simulink model "macroRobot_simulator"  (R2025a)
settings: Solver=FixedStepAuto  StartTime=0.0  StopTime=120  FixedStep=TsControl  MaxStep=0.00025  RelTol=1e-3
PreLoadFcn:
  | initMacroRobotSimulator;
InitFcn:
  | initMacroRobotSimulator;
values from neighbouring files (symbols this model uses):
  initState = deg2rad([-109; +67; +71; -111; -59; +20; -18])    [initMacroRobotSimulator.m]
undefined symbols (not defined in the file or in its folder): smiData, T_b_LaserGate, T_F1_Center, T_F1_Square1, T_F1_Square2, T_F1_Z1, T_F1_Z2, TsControl, X, Y, Z
libraries: sm_lib x50, nesl_utility x13, simulink x1, matrix_library x1, lib_lowLevelController x1, lib_ForwardKinematicsMacroRobot x1, lib_highLevelController x1, lib_InverseKinematicsMacroRobotVelocity x1, lib_saturateMacroRobotPosition x1
(part 2 of 2)

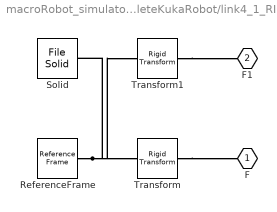
== system macroRobot_simulator/Simulation/completeKukaRobot/link4_1_RIGID ==
  ReferenceFrame : sm_lib/Frames and Transforms/Reference Frame
  Solid : sm_lib/Body Elements/File Solid  ExtGeomFileName=link4_Default_sldprt.STEP  UnitType=FromFile  ExtGeomFileUnits=m  StepReaderType=HEX  ExportConvexHullGeometry=off  InertiaType=Custom  BasedOnType=DensityFromFile  Density=1000  DensityUnits=kg/m^3  Mass=smiData.Solid(4).mass  MassUnits=kg  CenterOfMass=smiData.Solid(4).CoM  CenterOfMassUnits=mm  MomentsOfInertia=smiData.Solid(4).MoI  MomentsOfInertiaUnits=kg*mm^2  ProductsOfInertia=smiData.Solid(4).PoI  ProductsOfInertiaUnits=kg*mm^2  GraphicType=FromGeometry  MarkerShape=Sphere  MarkerSize=10  GraphicVisPropType=SimpleVisualProperties  GraphicDiffuseColor=smiData.Solid(4).color  GraphicOpacity=smiData.Solid(4).opacity  GraphicSpecularColor=[0.5 0.5 0.5 1.0]  GraphicAmbientColor=[0.15 0.15 0.15 1.0]  GraphicEmissiveColor=[0.0 0.0 0.0 1.0]  GraphicShininess=75  DoExposeReferenceFrame=on  SerializedFrames=<Frames/>
  Transform : sm_lib/Frames and Transforms/Rigid Transform  RotationMethod=ArbitraryAxis  FollAlignAxisA=+X  BaseAlignAxisA=+Y  FollAlignAxisB=+Y  BaseAlignAxisB=+Z  RotationStandardAxis=+Z  RotationAngle=smiData.RigidTransform(8).angle  RotationAngleUnits=rad  RotationArbitraryAxis=smiData.RigidTransform(8).axis  RotationSequenceAxes=FollowerAxes  RotationSequence=XYX  RotationSequenceAngles=[0 0 0]  RotationSequenceAnglesUnits=deg  RotationMatrix=[1 0 0; 0 1 0; 0 0 1]  Quaternion=[1 0 0 0]  TranslationMethod=Cartesian  TranslationCartesianOffset=smiData.RigidTransform(8).translation  TranslationCartesianOffsetUnits=mm  TranslationStandardAxis=+Z  TranslationStandardOffset=0  TranslationStandardOffsetUnits=m  TranslationROffset=0  TranslationROffsetUnits=m  TranslationThetaOffset=0  TranslationThetaOffsetUnits=deg  TranslationZOffset=0  TranslationZOffsetUnits=m
  Transform1 : sm_lib/Frames and Transforms/Rigid Transform  RotationMethod=ArbitraryAxis  FollAlignAxisA=+X  BaseAlignAxisA=+Y  FollAlignAxisB=+Y  BaseAlignAxisB=+Z  RotationStandardAxis=+Z  RotationAngle=smiData.RigidTransform(9).angle  RotationAngleUnits=rad  RotationArbitraryAxis=smiData.RigidTransform(9).axis  RotationSequenceAxes=FollowerAxes  RotationSequence=XYX  RotationSequenceAngles=[0 0 0]  RotationSequenceAnglesUnits=deg  RotationMatrix=[1 0 0; 0 1 0; 0 0 1]  Quaternion=[1 0 0 0]  TranslationMethod=Cartesian  TranslationCartesianOffset=smiData.RigidTransform(9).translation  TranslationCartesianOffsetUnits=mm  TranslationStandardAxis=+Z  TranslationStandardOffset=0  TranslationStandardOffsetUnits=m  TranslationROffset=0  TranslationROffsetUnits=m  TranslationThetaOffset=0  TranslationThetaOffsetUnits=deg  TranslationZOffset=0  TranslationZOffsetUnits=m
  F : PMIOPort  Side=Left
  F1 : PMIOPort  Port=2  Side=Right
  connections:
  ReferenceFrame/RConn1 -- Solid/RConn1 -- Transform/LConn1 -- Transform1/LConn1
  Transform/RConn1 -- F/RConn1
  Transform1/RConn1 -- F1/RConn1

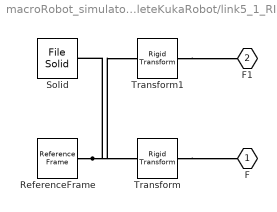
== system macroRobot_simulator/Simulation/completeKukaRobot/link5_1_RIGID ==
  ReferenceFrame : sm_lib/Frames and Transforms/Reference Frame
  Solid : sm_lib/Body Elements/File Solid  ExtGeomFileName=link5_Default_sldprt.STEP  UnitType=FromFile  ExtGeomFileUnits=m  StepReaderType=HEX  ExportConvexHullGeometry=off  InertiaType=Custom  BasedOnType=DensityFromFile  Density=1000  DensityUnits=kg/m^3  Mass=smiData.Solid(5).mass  MassUnits=kg  CenterOfMass=smiData.Solid(5).CoM  CenterOfMassUnits=mm  MomentsOfInertia=smiData.Solid(5).MoI  MomentsOfInertiaUnits=kg*mm^2  ProductsOfInertia=smiData.Solid(5).PoI  ProductsOfInertiaUnits=kg*mm^2  GraphicType=FromGeometry  MarkerShape=Sphere  MarkerSize=10  GraphicVisPropType=SimpleVisualProperties  GraphicDiffuseColor=smiData.Solid(5).color  GraphicOpacity=smiData.Solid(5).opacity  GraphicSpecularColor=[0.5 0.5 0.5 1.0]  GraphicAmbientColor=[0.15 0.15 0.15 1.0]  GraphicEmissiveColor=[0.0 0.0 0.0 1.0]  GraphicShininess=75  DoExposeReferenceFrame=on  SerializedFrames=<Frames/>
  Transform : sm_lib/Frames and Transforms/Rigid Transform  RotationMethod=ArbitraryAxis  FollAlignAxisA=+X  BaseAlignAxisA=+Y  FollAlignAxisB=+Y  BaseAlignAxisB=+Z  RotationStandardAxis=+Z  RotationAngle=smiData.RigidTransform(10).angle  RotationAngleUnits=rad  RotationArbitraryAxis=smiData.RigidTransform(10).axis  RotationSequenceAxes=FollowerAxes  RotationSequence=XYX  RotationSequenceAngles=[0 0 0]  RotationSequenceAnglesUnits=deg  RotationMatrix=[1 0 0; 0 1 0; 0 0 1]  Quaternion=[1 0 0 0]  TranslationMethod=Cartesian  TranslationCartesianOffset=smiData.RigidTransform(10).translation  TranslationCartesianOffsetUnits=mm  TranslationStandardAxis=+Z  TranslationStandardOffset=0  TranslationStandardOffsetUnits=m  TranslationROffset=0  TranslationROffsetUnits=m  TranslationThetaOffset=0  TranslationThetaOffsetUnits=deg  TranslationZOffset=0  TranslationZOffsetUnits=m
  Transform1 : sm_lib/Frames and Transforms/Rigid Transform  RotationMethod=ArbitraryAxis  FollAlignAxisA=+X  BaseAlignAxisA=+Y  FollAlignAxisB=+Y  BaseAlignAxisB=+Z  RotationStandardAxis=+Z  RotationAngle=smiData.RigidTransform(11).angle  RotationAngleUnits=rad  RotationArbitraryAxis=smiData.RigidTransform(11).axis  RotationSequenceAxes=FollowerAxes  RotationSequence=XYX  RotationSequenceAngles=[0 0 0]  RotationSequenceAnglesUnits=deg  RotationMatrix=[1 0 0; 0 1 0; 0 0 1]  Quaternion=[1 0 0 0]  TranslationMethod=Cartesian  TranslationCartesianOffset=smiData.RigidTransform(11).translation  TranslationCartesianOffsetUnits=mm  TranslationStandardAxis=+Z  TranslationStandardOffset=0  TranslationStandardOffsetUnits=m  TranslationROffset=0  TranslationROffsetUnits=m  TranslationThetaOffset=0  TranslationThetaOffsetUnits=deg  TranslationZOffset=0  TranslationZOffsetUnits=m
  F : PMIOPort  Side=Left
  F1 : PMIOPort  Port=2  Side=Right
  connections:
  ReferenceFrame/RConn1 -- Solid/RConn1 -- Transform/LConn1 -- Transform1/LConn1
  Transform/RConn1 -- F/RConn1
  Transform1/RConn1 -- F1/RConn1

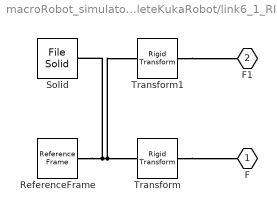
== system macroRobot_simulator/Simulation/completeKukaRobot/link6_1_RIGID ==
  ReferenceFrame : sm_lib/Frames and Transforms/Reference Frame
  Solid : sm_lib/Body Elements/File Solid  ExtGeomFileName=link6_Default_sldprt.STEP  UnitType=FromFile  ExtGeomFileUnits=m  StepReaderType=HEX  ExportConvexHullGeometry=off  InertiaType=Custom  BasedOnType=DensityFromFile  Density=1000  DensityUnits=kg/m^3  Mass=smiData.Solid(8).mass  MassUnits=kg  CenterOfMass=smiData.Solid(8).CoM  CenterOfMassUnits=mm  MomentsOfInertia=smiData.Solid(8).MoI  MomentsOfInertiaUnits=kg*mm^2  ProductsOfInertia=smiData.Solid(8).PoI  ProductsOfInertiaUnits=kg*mm^2  GraphicType=FromGeometry  MarkerShape=Sphere  MarkerSize=10  GraphicVisPropType=SimpleVisualProperties  GraphicDiffuseColor=smiData.Solid(8).color  GraphicOpacity=smiData.Solid(8).opacity  GraphicSpecularColor=[0.5 0.5 0.5 1.0]  GraphicAmbientColor=[0.15 0.15 0.15 1.0]  GraphicEmissiveColor=[0.0 0.0 0.0 1.0]  GraphicShininess=75  DoExposeReferenceFrame=on  SerializedFrames=<Frames/>
  Transform : sm_lib/Frames and Transforms/Rigid Transform  RotationMethod=ArbitraryAxis  FollAlignAxisA=+X  BaseAlignAxisA=+Y  FollAlignAxisB=+Y  BaseAlignAxisB=+Z  RotationStandardAxis=+Z  RotationAngle=smiData.RigidTransform(12).angle  RotationAngleUnits=rad  RotationArbitraryAxis=smiData.RigidTransform(12).axis  RotationSequenceAxes=FollowerAxes  RotationSequence=XYX  RotationSequenceAngles=[0 0 0]  RotationSequenceAnglesUnits=deg  RotationMatrix=[1 0 0; 0 1 0; 0 0 1]  Quaternion=[1 0 0 0]  TranslationMethod=Cartesian  TranslationCartesianOffset=smiData.RigidTransform(12).translation  TranslationCartesianOffsetUnits=mm  TranslationStandardAxis=+Z  TranslationStandardOffset=0  TranslationStandardOffsetUnits=m  TranslationROffset=0  TranslationROffsetUnits=m  TranslationThetaOffset=0  TranslationThetaOffsetUnits=deg  TranslationZOffset=0  TranslationZOffsetUnits=m
  Transform1 : sm_lib/Frames and Transforms/Rigid Transform  RotationMethod=ArbitraryAxis  FollAlignAxisA=+X  BaseAlignAxisA=+Y  FollAlignAxisB=+Y  BaseAlignAxisB=+Z  RotationStandardAxis=+Z  RotationAngle=smiData.RigidTransform(13).angle  RotationAngleUnits=rad  RotationArbitraryAxis=smiData.RigidTransform(13).axis  RotationSequenceAxes=FollowerAxes  RotationSequence=XYX  RotationSequenceAngles=[0 0 0]  RotationSequenceAnglesUnits=deg  RotationMatrix=[1 0 0; 0 1 0; 0 0 1]  Quaternion=[1 0 0 0]  TranslationMethod=Cartesian  TranslationCartesianOffset=smiData.RigidTransform(13).translation  TranslationCartesianOffsetUnits=mm  TranslationStandardAxis=+Z  TranslationStandardOffset=0  TranslationStandardOffsetUnits=m  TranslationROffset=0  TranslationROffsetUnits=m  TranslationThetaOffset=0  TranslationThetaOffsetUnits=deg  TranslationZOffset=0  TranslationZOffsetUnits=m
  F : PMIOPort  Side=Left
  F1 : PMIOPort  Port=2  Side=Right
  connections:
  ReferenceFrame/RConn1 -- Transform/LConn1 -- Transform1/LConn1 -- Solid/RConn1
  Transform/RConn1 -- F/RConn1
  Transform1/RConn1 -- F1/RConn1

== system macroRobot_simulator/Simulation/completeKukaRobot/link7_1_RIGID ==
  ReferenceFrame : sm_lib/Frames and Transforms/Reference Frame
  Solid : sm_lib/Body Elements/File Solid  ExtGeomFileName=link7_Default_sldprt.STEP  UnitType=FromFile  ExtGeomFileUnits=m  StepReaderType=HEX  ExportConvexHullGeometry=off  InertiaType=Custom  BasedOnType=DensityFromFile  Density=1000  DensityUnits=kg/m^3  Mass=smiData.Solid(1).mass  MassUnits=kg  CenterOfMass=smiData.Solid(1).CoM  CenterOfMassUnits=mm  MomentsOfInertia=smiData.Solid(1).MoI  MomentsOfInertiaUnits=kg*mm^2  ProductsOfInertia=smiData.Solid(1).PoI  ProductsOfInertiaUnits=kg*mm^2  GraphicType=FromGeometry  MarkerShape=Sphere  MarkerSize=10  GraphicVisPropType=SimpleVisualProperties  GraphicDiffuseColor=smiData.Solid(1).color  GraphicOpacity=smiData.Solid(1).opacity  GraphicSpecularColor=[0.5 0.5 0.5 1.0]  GraphicAmbientColor=[0.15 0.15 0.15 1.0]  GraphicEmissiveColor=[0.0 0.0 0.0 1.0]  GraphicShininess=75  DoExposeReferenceFrame=on  SerializedFrames=<Frames><Frame><Id>Frame1</Id><Value><Name>F1</Name><Origin><Source>GeometricFeature</Source><FeatureName>planar surface 30</FeatureName></Origin><PrimaryAxis><DefinedDirection>+Z</DefinedDirection><Source>ReferenceFrame</Source><SourceDirection>+Z</SourceDirection><FeatureName></FeatureName></PrimaryAxis><SecondaryAxis><DefinedDirection>+X</DefinedDirection><Source>ReferenceFrame</Source><SourceDirection>+X</SourceDirection><FeatureName></FeatureName></SecondaryAxis></Value></Frame></Frames>
  Transform : sm_lib/Frames and Transforms/Rigid Transform  RotationMethod=ArbitraryAxis  FollAlignAxisA=+X  BaseAlignAxisA=+Y  FollAlignAxisB=+Y  BaseAlignAxisB=+Z  RotationStandardAxis=+Z  RotationAngle=smiData.RigidTransform(14).angle  RotationAngleUnits=rad  RotationArbitraryAxis=smiData.RigidTransform(14).axis  RotationSequenceAxes=FollowerAxes  RotationSequence=XYX  RotationSequenceAngles=[0 0 0]  RotationSequenceAnglesUnits=deg  RotationMatrix=[1 0 0; 0 1 0; 0 0 1]  Quaternion=[1 0 0 0]  TranslationMethod=Cartesian  TranslationCartesianOffset=smiData.RigidTransform(14).translation  TranslationCartesianOffsetUnits=mm  TranslationStandardAxis=+Z  TranslationStandardOffset=0  TranslationStandardOffsetUnits=m  TranslationROffset=0  TranslationROffsetUnits=m  TranslationThetaOffset=0  TranslationThetaOffsetUnits=deg  TranslationZOffset=0  TranslationZOffsetUnits=m
  F : PMIOPort  Side=Left
  F1 : PMIOPort  Port=2  Side=Right
  connections:
  ReferenceFrame/RConn1 -- Solid/RConn1 -- Transform/LConn1
  Transform/RConn1 -- F/RConn1
  F1/RConn1 -- Solid/LConn1

== system macroRobot_simulator/Simulation/completeKukaRobot/tool ==
  File Solid : sm_lib/Body Elements/File Solid  ExtGeomFileName=/home/gordi/Documentos/Máster/BASILEA/3rd Semester/A. Medical Robotics/Project/codeBaseSimulator/Library/Visualizer/20261016_extruder_mockup.STEP  UnitType=FromFile  ExtGeomFileUnits=m  StepReaderType=HEX  ExportConvexHullGeometry=off  InertiaType=PointMass  BasedOnType=DensityFromFile  Density=1000  DensityUnits=kg/m^3  Mass=1  MassUnits=kg  CenterOfMass=[0 0 0]  CenterOfMassUnits=m  MomentsOfInertia=[1 1 1]  MomentsOfInertiaUnits=kg*m^2  ProductsOfInertia=[0 0 0]  ProductsOfInertiaUnits=kg*m^2  GraphicType=FromGeometry  MarkerShape=Sphere  MarkerSize=10  GraphicVisPropType=SimpleVisualProperties  GraphicDiffuseColor=[0.5 0.5 0.5]  GraphicOpacity=1  GraphicSpecularColor=[0.5 0.5 0.5 1.0]  GraphicAmbientColor=[0.15 0.15 0.15 1.0]  GraphicEmissiveColor=[0.0 0.0 0.0 1.0]  GraphicShininess=75  DoExposeReferenceFrame=off  SerializedFrames=<Frames><Frame><Id>Frame1</Id><Value><Name>F1</Name><Origin><Source>GeometricFeature</Source><FeatureName>planar surface 33</FeatureName></Origin><PrimaryAxis><DefinedDirection>-Z</DefinedDirection><Source>GeometricFeature</Source><SourceDirection>+Y</SourceDirection><FeatureName>segment 40</FeatureName></PrimaryAxis><SecondaryAxis><DefinedDirection>+X</DefinedDirection><Source>GeometricFeature</Source><SourceDirection>+Z</SourceDirection><FeatureName>segment 53</FeatureName></SecondaryAxis></Value></Frame><Frame><Id>Frame2</Id><Value><Name>F2</Name><Origin><Source>GeometricFeature</Source><FeatureName>planar surface 266</FeatureName></Origin><PrimaryAxis><DefinedDirection>+Z</DefinedDirection><Source>ReferenceFrame</Source><SourceDirection>-Y</SourceDirection><FeatureName></FeatureName></PrimaryAxis><SecondaryAxis><DefinedDirection>+X</DefinedDirection><Source>ReferenceFrame</Source><SourceDirection>-Z</SourceDirection><FeatureName></FeatureName></SecondaryAxis></Value></Frame></Frames>
  ReferenceFrame : sm_lib/Frames and Transforms/Reference Frame
  Transform1 : sm_lib/Frames and Transforms/Rigid Transform  Commented=on  RotationMethod=RotationMatrix  FollAlignAxisA=+X  BaseAlignAxisA=+Y  FollAlignAxisB=+Y  BaseAlignAxisB=+Z  RotationStandardAxis=+Z  RotationAngle=smiData.RigidTransform(14).angle  RotationAngleUnits=rad  RotationArbitraryAxis=smiData.RigidTransform(14).axis  RotationSequenceAxes=FollowerAxes  RotationSequence=XYX  RotationSequenceAngles=[0 0 0]  RotationSequenceAnglesUnits=deg  RotationMatrix=[cos(pi/4) 0 -sin(pi/4); 0 1 0; sin(pi/4) 0 cos(pi/4)]  Quaternion=[1 0 0 0]  TranslationMethod=Cartesian  TranslationCartesianOffset=[0.0462 0 0.1452]  TranslationCartesianOffsetUnits=mm  TranslationStandardAxis=+Z  TranslationStandardOffset=0  TranslationStandardOffsetUnits=m  TranslationROffset=0  TranslationROffsetUnits=m  TranslationThetaOffset=0  TranslationThetaOffsetUnits=deg  TranslationZOffset=0  TranslationZOffsetUnits=m
  F1 : PMIOPort  Side=Left
  F2 : PMIOPort  Port=2  Side=Right
  connections:
  ReferenceFrame/RConn1 -- F1/RConn1 -- File Solid/LConn1
  File Solid/RConn1 -- F2/RConn1

== matlab function macroRobot_simulator/Simulation/completeKukaRobot/MATLAB Function ==
  data: commandedJoints input; jointsForModel output
function jointsForModel  = jointOrientationToModel(commandedJoints)


jointsForModel = commandedJoints(1:7);
jointsForModel([3,4,5,6,7]) = -commandedJoints([3,4,5,6,7]);
%joints(5) = -u(5);
end

== matlab function macroRobot_simulator/Controller/MATLAB Function rotPos2Trasnform ==
  data: pos input; ori input; T_base_tcp output
function T_base_tcp = rotPos2Transform(pos, ori)

T_base_tcp = eye(4); % Identity matrix
T_base_tcp(1:3,4) = pos;
T_base_tcp(1:3,1:3) = ori;

== matlab function macroRobot_simulator/Simulation/calibrationGate/laserGate/MATLAB Function ==
  data: R input; p input; T output
function T = posRot2Transform(R, p)
    T = eye(4);
    T(1:3, 1:3) = R;
    T(1:3, 4) = p;
end

== stateflow chart macroRobot_simulator/Controller/CalibrationSequence ==
  state StartCalibration
    codeState = -1;
    codeVel = 0;
    T_F1_des = T_F1_Center;
    counter = 0;
  state VertexA
    codeState = 0;
    codeVel = 0;
    T_F1_des = T_F1_Square1(:,:,1);
  state CalibrationPlane1
    codeState = 1;
    codeVel = 1;
    state VertexA
      T_F1_des = T_F1_Square1(:,:,1);
    state VertexD
      T_F1_des = T_F1_Square1(:,:,4);
    state VertexC
      T_F1_des = T_F1_Square1(:,:,3);
    state VertexB
      T_F1_des = T_F1_Square1(:,:,2);
    CalibrationPlane1.VertexD -> CalibrationPlane1.VertexA : [trigger==1&&...
        | counter==3]
        | {counter = 4;}
    CalibrationPlane1.VertexC -> CalibrationPlane1.VertexD : [trigger== 1&&...
        | counter==2]
        | {counter = 3;}
    (default) -> CalibrationPlane1.VertexB
    CalibrationPlane1.VertexB -> CalibrationPlane1.VertexC : [trigger== 1&&...
        | counter==1]
        | {counter = 2;}
  state CalibrationPlane2
    codeState = 2;
    codeVel = 1;
    state VertexA
      T_F1_des = T_F1_Square2(:,:,1);
    state VertexD
      T_F1_des = T_F1_Square2(:,:,4);
    state VertexC
      T_F1_des = T_F1_Square2(:,:,3);
    state VertexB
      T_F1_des = T_F1_Square2(:,:,2);
    (default) -> CalibrationPlane2.VertexA
    CalibrationPlane2.VertexD -> CalibrationPlane2.VertexA : [trigger==1&&...
        | counter==3]
        | {counter = 4;}
    CalibrationPlane2.VertexC -> CalibrationPlane2.VertexD : [trigger== 1&&...
        | counter==2]
        | {counter = 3;}
    CalibrationPlane2.VertexA -> CalibrationPlane2.VertexB [order 1] : [trigger==1&&...
        | counter==0]
        | {counter = 1;}
    CalibrationPlane2.VertexB -> CalibrationPlane2.VertexC : [trigger== 1&&...
        | counter==1]
        | {counter = 2;}
  state BackToInit
    codeVel = 0;
    T_F1_des = T_F1_Center;
    codeState = 0;
  state CalibrationPlane3
    codeState = 3;
    codeVel = 1;
    state VertexA
      T_F1_des = T_F1_Square2(:,:,1);
    state VertexD
      T_F1_des = T_F1_Square2(:,:,4);
    state VertexC
      T_F1_des = T_F1_Square2(:,:,3);
    state VertexB
      T_F1_des = T_F1_Square2(:,:,2);
    (default) -> CalibrationPlane3.VertexA
    CalibrationPlane3.VertexD -> CalibrationPlane3.VertexA : [trigger==1&&...
        | counter==3]
        | {counter = 4;}
    CalibrationPlane3.VertexC -> CalibrationPlane3.VertexD : [trigger== 1&&...
        | counter==2]
        | {counter = 3;}
    CalibrationPlane3.VertexA -> CalibrationPlane3.VertexB : [trigger==1&&...
        | counter==0]
        | {counter = 1;}
    CalibrationPlane3.VertexB -> CalibrationPlane3.VertexC : [trigger== 1&&...
        | counter==1]
        | {counter = 2;}
  state CalibrationZ
    codeState = 5;
    state AbovePlane
      T_F1_des = T_F1_Z1;
    state CrossPlane
      T_F1_des = T_F1_Z2;
    (default) -> AbovePlane : [calibOK == 1]
    AbovePlane -> CrossPlane : [trigger==1]
  (default) -> StartCalibration
  StartCalibration -> VertexA : [after(0.2, sec) && trigger == 1]
  VertexA -> CalibrationPlane1 : [trigger==1&&counter==0]
      | {counter = 1;}
  CalibrationPlane1.VertexA -> CalibrationPlane2 : [trigger==1&&...
      | counter==4]
      | {counter = 0;}
  CalibrationPlane2.VertexA -> BackToInit [order 2] : [trigger==1&&...
      | counter==4]
      | {counter = 0}
  BackToInit -> CalibrationPlane3 : [trigger==1 && counter==0 && calibOK == 1 ]
  CalibrationPlane3 -> CalibrationZ : [trigger==1&&...
      | counter==4]
      | {counter = 0}
  data: T_F1_Center parameter; T_F1_des output; counter local; trigger input; T_F1_Square1 parameter; T_F1_Square2 parameter; T_F1_Z1 parameter; T_F1_Z2 parameter; codeVel output; codeState output; calibOK input

== matlab function macroRobot_simulator/Simulation/MATLAB Function ==
  data: p input; triggerX output; triggerY output
function [triggerX, triggerY] = laserTrigger(p)
    
    thickness = 12e-3;
    tolerance = 5e-4;
    triggerX = 0;
    triggerY = 0;

    if abs(p(3)) < thickness
        if abs(p(1)) < tolerance
            triggerX = 1;
        elseif abs(p(2)) < tolerance
            triggerY = 1;
        end
    end
    
end

== matlab function macroRobot_simulator/Controller/MATLAB Function ==
  data: plane_X output; plane_Y output; laserX input; laserY input; T_base_tcp input; plane_X input; plane_Y input; triggerX input; triggerY input; triggerX output; triggerY output; codeState input
function [plane_X, plane_Y, triggerX, triggerY] = capturePoses(laserX, laserY, T_base_tcp, plane_X, plane_Y, triggerX, triggerY, codeState)
[plane_X, plane_Y, triggerX, triggerY] = fun_capturePoses(laserX, laserY, T_base_tcp, plane_X, plane_Y, triggerX, triggerY, codeState);

== matlab function macroRobot_simulator/Controller/MATLAB Function1 ==
  data: deltasX output; deltasY output; Rd output; Y input; X input; calibOK output size=1; codeState input; offset parameter
function [deltasX, deltasY, Rd, calibOK]  = calibrate(Y, X, codeState, offset)
[deltasX, deltasY, Rd, calibOK] = fun_calibrate(Y, X, codeState, offset);
